simulink model "final2q_all_cases"  (R2024b)
settings: Solver=VariableStepAuto  StartTime=0.0  StopTime=10  RelTol=1e-3
undefined symbols (not defined in the file): Down, Up
libraries: spsSeriesRLCBranchLib x30, spsDCVoltageSourceLib x12, spsIGBTDiodeLib x12, spsVoltageMeasurementLib x12, spsCurrentMeasurementLib x6, slpidlib x2, eePwmGenerator x2, sps_lib x1
settings Model: Creator=jmy  LastModifiedBy=Eng.Abd-Elrhman Saad

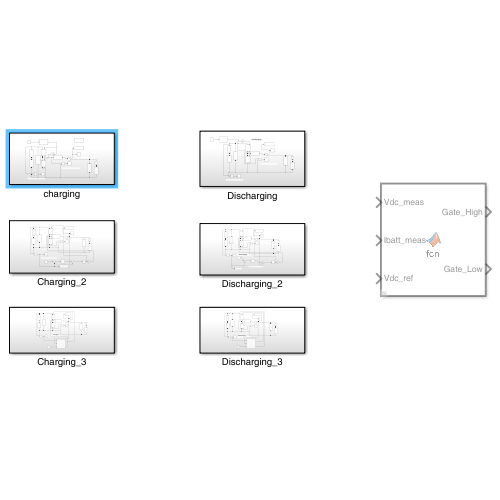
[thumbnail: Simulink's stored preview of the top-level diagram]
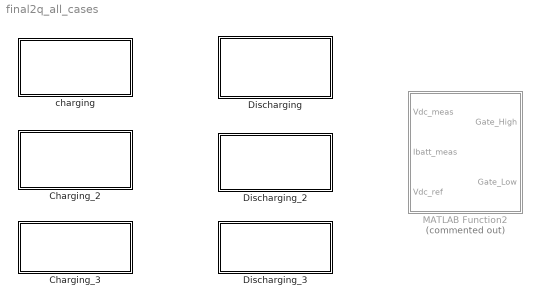
== system final2q_all_cases ==
  Charging_2 : Subsystem
  Charging_3 : Subsystem
  Discharging : Subsystem
  Discharging_2 : Subsystem
  Discharging_3 : Subsystem
  MATLAB Function2 : MATLAB Function  Commented=on  TreatAsAtomicUnit=on
  charging : Subsystem

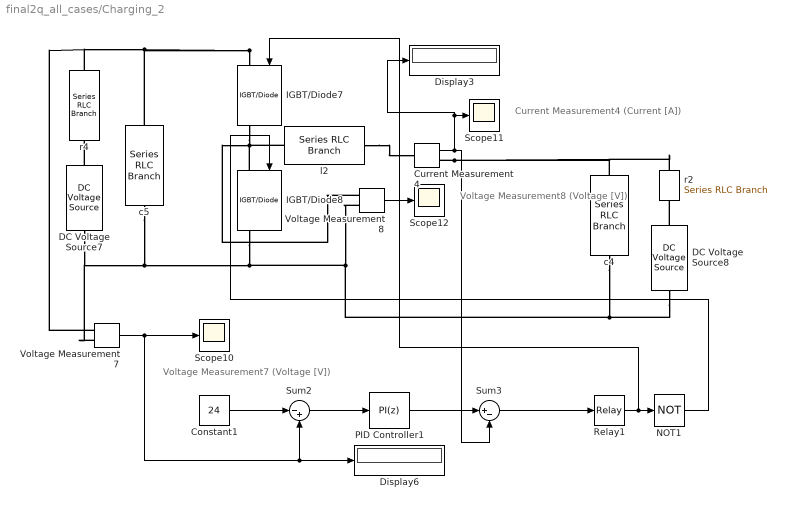
== system final2q_all_cases/Charging_2 ==
  note: Voltage Measurement7 (Voltage [V])
  note: Current Measurement4 (Current [A])
  note: Voltage Measurement8 (Voltage [V])
  Constant1 : Constant  Value=24
  Current Measurement4 : spsCurrentMeasurementLib/Current Measurement  PhasorSimulation=off  OutputType=Complex  PSBequivalent=0
  DC Voltage Source7 : spsDCVoltageSourceLib/DC Voltage Source  Amplitude=26  Measurements=None
  DC Voltage Source8 : spsDCVoltageSourceLib/DC Voltage Source  Amplitude=18.5  Measurements=None
  Display3 : Display
  Display6 : Display
  IGBT/Diode7 : spsIGBTDiodeLib/IGBT//Diode  Ron=1e-3  Rs=1e5  Cs=inf  Measurements=on
  IGBT/Diode8 : spsIGBTDiodeLib/IGBT//Diode  Ron=1e-3  Rs=1e5  Cs=inf  Measurements=on
  NOT1 : Logic  Operator=NOT  IconShape=distinctive  AllPortsSameDT=off  OutDataTypeStr=boolean
  PID Controller1 : slpidlib/PID Controller  Controller=PI  Form=Parallel  TimeDomain=Discrete-time  UseExternalTs=off  SampleTime=-1  IntegratorMethod=Forward Euler  FilterMethod=Forward Euler  ControllerParametersSource=internal  P=0.1  I=10  UseKiTs=off  D=0  UseExternalDerivativeSource=off  N=100  UseFilter=on  TunerSelectOption=Transfer Function Based (PID Tuner App)  InitialConditionSource=internal  InitialConditionForIntegrator=0  InitialConditionForFilter=0  DifferentiatorICPrevScaledInput=0  ExternalReset=none  TrackingMode=off  Kt=1  LimitOutput=on  SatLimitsSource=internal  UpperSaturationLimit=3.1  LowerSaturationLimit=-10  LinearizeAsGain=off  AntiWindupMode=none  Kb=1  LimitIntegrator=off  UpperIntegratorSaturationLimit=inf  LowerIntegratorSaturationLimit=-inf  POutMin=[]  POutMax=[]  IOutMin=[]  IOutMax=[]  DOutMin=[]  DOutMax=[]  NOutMin=[]  NOutMax=[]  SumOutMin=[]  SumOutMax=[]  SaturationOutMin=[]  SaturationOutMax=[]  PParamMin=[]  PParamMax=[]  IParamMin=[]  IParamMax=[]  DParamMin=[]  DParamMax=[]  NParamMin=[]  NParamMax=[]  KbParamMin=[]  KbParamMax=[]  KtParamMin=[]  KtParamMax=[]  KbOutMin=[]  KbOutMax=[]  KtOutMin=[]  KtOutMax=[]  IntegratorOutMin=[]  IntegratorOutMax=[]  FilterOutMin=[]  FilterOutMax=[]  SumI1OutMin=[]  SumI1OutMax=[]  SumI2OutMin=[]  SumI2OutMax=[]  SumI3OutMin=[]  SumI3OutMax=[]  SumI4OutMin=[]  SumI4OutMax=[]  SumDOutMin=[]  SumDOutMax=[]  DifferentiatorOutMin=[]  DifferentiatorOutMax=[]  FilterDiffOutCoefMin=[]  FilterDiffOutCoefMax=[]  ReciprocalOutMin=[]  ReciprocalOutMax=[]  SumDenOutMin=[]  SumDenOutMax=[]  SumNumOutMin=[]  SumNumOutMax=[]  DivideOutMin=[]  DivideOutMax=[]  UdiffTsProdOutMin=[]  UdiffTsProdOutMax=[]  NTsProdOutMin=[]  NTsProdOutMax=[]  UintegralTsProdOutMin=[]  UintegralTsProdOutMax=[]  UngainTsProdOutMin=[]  UngainTsProdOutMax=[]  ClampingZeroOutDataTypeStr=Inherit: Inherit via back propagation  ClampingZeroOutMin=[]  ClampingZeroOutMax=[]  FilterDenConstantOutDataTypeStr=Inherit: Inherit via back propagation  FilterDenConstantOutMin=[]  FilterDenConstantOutMax=[]  PCopyOutDataTypeStr=Inherit: Inherit via back propagation  PCopyOutMin=[]  PCopyOutMax=[]  NCopyOutDataTypeStr=Inherit: Inherit via back propagation  NCopyOutMin=[]  NCopyOutMax=[]  IntegratorContinuousStateAttributes=''  IntegratorStateMustResolveToSignalObject=off  IntegratorRTWStateStorageClass=Auto  FilterContinuousStateAttributes=''  FilterStateMustResolveToSignalObject=off  FilterRTWStateStorageClass=Auto  ParallelPVariant=InternalParameters  IdealPVariant=Disabled  IVariant=InternalParameters  DVariant=Disabled  IntegratorVariant=Discrete  SatVariant=Enabled  AWVariant=Passthrough  PCopyVariant=Disabled  TRVariant=Disabled  FdbkBlocksVariant=Forward  IdealPFdbkVariant=Disabled  SatFdbkVariant=Disabled  DerivativeFilterVariant=Disabled  NVariant=Disabled  NCopyVariant=Disabled_SignalSpec  FilterICVariant=Disabled  IntegratorICVariant=InternalICs  ExternalResetVariant=Disabled  TRSumVariant=Passthrough  SumFdbkVariant=Disabled  SumVariant=Sum_PI  TsampFilterVariant=InternalTs  TsampNgainVariant=Passthrough  TsampIntegralVariant=Disabled_SignalSpec  ExternalSaturationOutDataTypeStr=Inherit: Same as second input  DerivativeSourceVariant=Disabled  PreIntVariant=InternalPreInt
  Relay1 : Relay  OnSwitchValue=0.5  OffSwitchValue=-0.5
  Scope10 : Scope
  Scope11 : Scope
  Scope12 : Scope
  Sum2 : Sum  Inputs=|-+
  Sum3 : Sum  Inputs=|+-
  Voltage Measurement7 : spsVoltageMeasurementLib/Voltage Measurement  PhasorSimulation=off  OutputType=Complex  PSBequivalent=0
  Voltage Measurement8 : spsVoltageMeasurementLib/Voltage Measurement  PhasorSimulation=off  OutputType=Complex  PSBequivalent=0
  c4 : spsSeriesRLCBranchLib/Series RLC Branch  LConnTagsString=__new0  RConnTagsString=__new0  BranchType=C  Resistance=1  Inductance=400e-6  SetiL0=off  InitialCurrent=0  Capacitance=100e-6  Setx0=off  InitialVoltage=0  Measurements=None
  c5 : spsSeriesRLCBranchLib/Series RLC Branch  LConnTagsString=__new0  RConnTagsString=__new0  BranchType=C  Resistance=1  Inductance=400e-6  SetiL0=off  InitialCurrent=0  Capacitance=220e-6  Setx0=off  InitialVoltage=0  Measurements=None
  l2 : spsSeriesRLCBranchLib/Series RLC Branch  LConnTagsString=__new0  RConnTagsString=__new0  BranchType=L  Resistance=1  Inductance=400e-6  SetiL0=off  InitialCurrent=0  Capacitance=1e-6  Setx0=off  InitialVoltage=0  Measurements=None
  r2 : spsSeriesRLCBranchLib/Series RLC Branch  LConnTagsString=__new0  RConnTagsString=__new0  BranchType=R  Resistance=0.0001  Inductance=400e-6  SetiL0=off  InitialCurrent=0  Capacitance=220e-6  Setx0=off  InitialVoltage=0  Measurements=None
  r4 : spsSeriesRLCBranchLib/Series RLC Branch  LConnTagsString=__new0  RConnTagsString=__new0  BranchType=R  Resistance=0.0001  Inductance=400e-6  SetiL0=off  InitialCurrent=0  Capacitance=220e-6  Setx0=off  InitialVoltage=0  Measurements=None
  wires:
  Voltage Measurement7/1 -> Scope10/1, Sum2/2, Display6/1
  Relay1/1 -> NOT1/1, IGBT/Diode7/1
  Voltage Measurement8/1 -> Scope12/1
  Constant1/1 -> Sum2/1
  Current Measurement4/1 -> Sum3/2, Display3/1, Scope11/1
  Sum3/1 -> Relay1/1
  NOT1/1 -> IGBT/Diode8/1
  Sum2/1 -> PID Controller1/1
  PID Controller1/1 -> Sum3/1
  connections:
  IGBT/Diode7/LConn1 -- r4/LConn1 -- Voltage Measurement7/LConn1 -- c5/LConn1
  DC Voltage Source8/LConn1 -- c4/RConn1 -- Voltage Measurement8/LConn2 -- Voltage Measurement7/LConn2 -- DC Voltage Source7/LConn1 -- c5/RConn1 -- IGBT/Diode8/RConn1
  DC Voltage Source8/RConn1 -- r2/RConn1
  l2/LConn1 -- IGBT/Diode8/LConn1 -- IGBT/Diode7/RConn1 -- Voltage Measurement8/LConn1
  Current Measurement4/RConn1 -- r2/LConn1 -- c4/LConn1
  l2/RConn1 -- Current Measurement4/LConn1
  DC Voltage Source7/RConn1 -- r4/RConn1

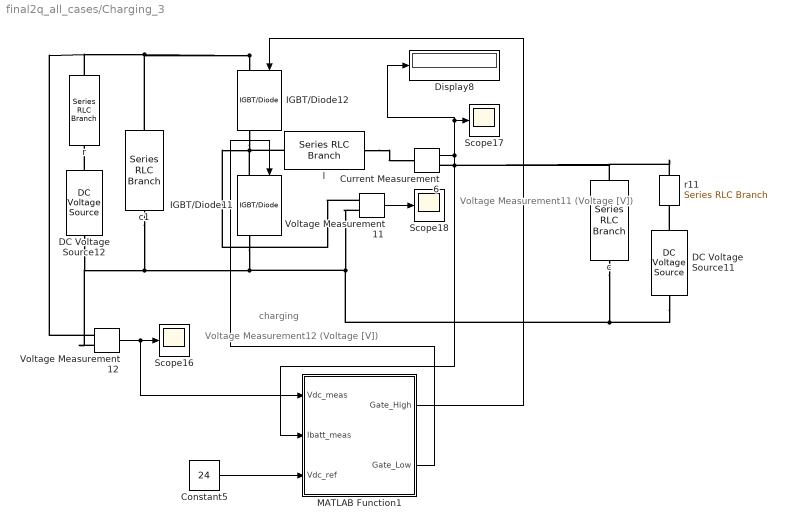
== system final2q_all_cases/Charging_3 ==
  note: charging
  note: Voltage Measurement12 (Voltage [V])
  note: Voltage Measurement11 (Voltage [V])
  Constant5 : Constant  Value=24
  Current Measurement6 : spsCurrentMeasurementLib/Current Measurement  PhasorSimulation=off  OutputType=Complex  PSBequivalent=0
  DC Voltage Source11 : spsDCVoltageSourceLib/DC Voltage Source  Amplitude=18.5  Measurements=None
  DC Voltage Source12 : spsDCVoltageSourceLib/DC Voltage Source  Amplitude=26  Measurements=None
  Display8 : Display
  IGBT/Diode11 : spsIGBTDiodeLib/IGBT//Diode  Ron=1e-3  Rs=1e5  Cs=inf  Measurements=on
  IGBT/Diode12 : spsIGBTDiodeLib/IGBT//Diode  Ron=1e-3  Rs=1e5  Cs=inf  Measurements=on
  MATLAB Function1 : MATLAB Function  TreatAsAtomicUnit=on
  Scope16 : Scope
  Scope17 : Scope
  Scope18 : Scope
  Voltage Measurement11 : spsVoltageMeasurementLib/Voltage Measurement  PhasorSimulation=off  OutputType=Complex  PSBequivalent=0
  Voltage Measurement12 : spsVoltageMeasurementLib/Voltage Measurement  PhasorSimulation=off  OutputType=Complex  PSBequivalent=0
  c : spsSeriesRLCBranchLib/Series RLC Branch  LConnTagsString=__new0  RConnTagsString=__new0  BranchType=C  Resistance=1  Inductance=400e-6  SetiL0=off  InitialCurrent=0  Capacitance=100e-6  Setx0=off  InitialVoltage=0  Measurements=None
  c1 : spsSeriesRLCBranchLib/Series RLC Branch  LConnTagsString=__new0  RConnTagsString=__new0  BranchType=C  Resistance=1  Inductance=400e-6  SetiL0=off  InitialCurrent=0  Capacitance=220e-6  Setx0=off  InitialVoltage=0  Measurements=None
  l : spsSeriesRLCBranchLib/Series RLC Branch  LConnTagsString=__new0  RConnTagsString=__new0  BranchType=L  Resistance=1  Inductance=400e-6  SetiL0=off  InitialCurrent=0  Capacitance=1e-6  Setx0=off  InitialVoltage=0  Measurements=None
  r : spsSeriesRLCBranchLib/Series RLC Branch  LConnTagsString=__new0  RConnTagsString=__new0  BranchType=R  Resistance=0.0001  Inductance=400e-6  SetiL0=off  InitialCurrent=0  Capacitance=220e-6  Setx0=off  InitialVoltage=0  Measurements=None
  r11 : spsSeriesRLCBranchLib/Series RLC Branch  LConnTagsString=__new0  RConnTagsString=__new0  BranchType=R  Resistance=0.0001  Inductance=400e-6  SetiL0=off  InitialCurrent=0  Capacitance=220e-6  Setx0=off  InitialVoltage=0  Measurements=None
  wires:
  Constant5/1 -> MATLAB Function1/3(Vdc_ref)
  Voltage Measurement12/1 -> Scope16/1, MATLAB Function1/1(Vdc_meas)
  MATLAB Function1/2(Gate_Low) -> IGBT/Diode11/1
  MATLAB Function1/1(Gate_High) -> IGBT/Diode12/1
  Current Measurement6/1 -> MATLAB Function1/2(Ibatt_meas), Display8/1, Scope17/1
  Voltage Measurement11/1 -> Scope18/1
  connections:
  IGBT/Diode12/LConn1 -- r/LConn1 -- Voltage Measurement12/LConn1 -- c1/LConn1
  DC Voltage Source11/LConn1 -- Voltage Measurement12/LConn2 -- DC Voltage Source12/LConn1 -- c1/RConn1 -- IGBT/Diode11/RConn1 -- Voltage Measurement11/LConn2 -- c/RConn1
  DC Voltage Source12/RConn1 -- r/RConn1
  Current Measurement6/RConn1 -- r11/LConn1 -- c/LConn1
  l/LConn1 -- IGBT/Diode11/LConn1 -- IGBT/Diode12/RConn1 -- Voltage Measurement11/LConn1
  l/RConn1 -- Current Measurement6/LConn1
  DC Voltage Source11/RConn1 -- r11/RConn1

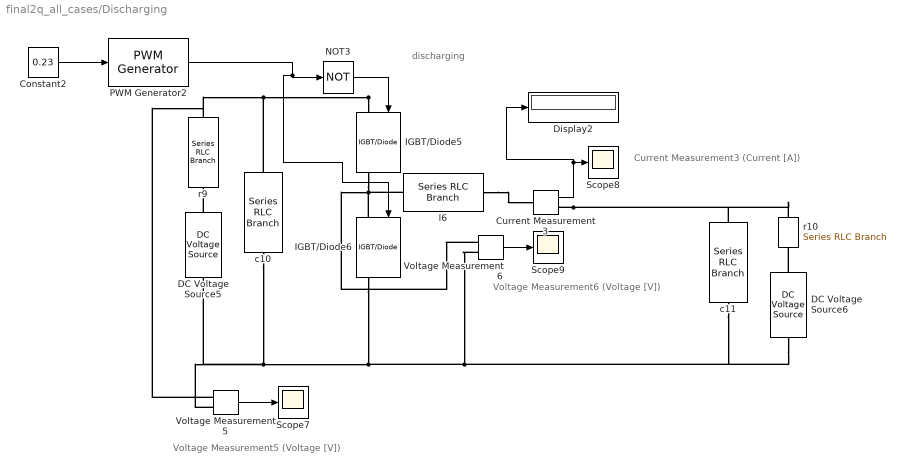
== system final2q_all_cases/Discharging ==
  note: discharging
  note: Voltage Measurement5 (Voltage [V])
  note: Current Measurement3 (Current [A])
  note: Voltage Measurement6 (Voltage [V])
  Constant2 : Constant  Value=0.23
  Current Measurement3 : spsCurrentMeasurementLib/Current Measurement  PhasorSimulation=off  OutputType=Complex  PSBequivalent=0
  DC Voltage Source5 : spsDCVoltageSourceLib/DC Voltage Source  Amplitude=22  Measurements=None
  DC Voltage Source6 : spsDCVoltageSourceLib/DC Voltage Source  Amplitude=18.5  Measurements=None
  Display2 : Display
  IGBT/Diode5 : spsIGBTDiodeLib/IGBT//Diode  Ron=1e-3  Rs=1e5  Cs=inf  Measurements=on
  IGBT/Diode6 : spsIGBTDiodeLib/IGBT//Diode  Ron=1e-3  Rs=1e5  Cs=inf  Measurements=on
  NOT3 : Logic  Operator=NOT  IconShape=distinctive  AllPortsSameDT=off  OutDataTypeStr=boolean
  PWM Generator2 : eePwmGenerator/PWM Generator  CarrCount=Up-Down  Tper=0.001  Tdelay=0  Ts=5e-5
  Scope7 : Scope
  Scope8 : Scope
  Scope9 : Scope
  Voltage Measurement5 : spsVoltageMeasurementLib/Voltage Measurement  PhasorSimulation=off  OutputType=Complex  PSBequivalent=0
  Voltage Measurement6 : spsVoltageMeasurementLib/Voltage Measurement  PhasorSimulation=off  OutputType=Complex  PSBequivalent=0
  c10 : spsSeriesRLCBranchLib/Series RLC Branch  LConnTagsString=__new0  RConnTagsString=__new0  BranchType=C  Resistance=1  Inductance=400e-6  SetiL0=off  InitialCurrent=0  Capacitance=220e-6  Setx0=off  InitialVoltage=0  Measurements=None
  c11 : spsSeriesRLCBranchLib/Series RLC Branch  LConnTagsString=__new0  RConnTagsString=__new0  BranchType=C  Resistance=1  Inductance=400e-6  SetiL0=off  InitialCurrent=0  Capacitance=100e-6  Setx0=off  InitialVoltage=0  Measurements=None
  l6 : spsSeriesRLCBranchLib/Series RLC Branch  LConnTagsString=__new0  RConnTagsString=__new0  BranchType=L  Resistance=1  Inductance=400e-6  SetiL0=off  InitialCurrent=0  Capacitance=1e-6  Setx0=off  InitialVoltage=0  Measurements=None
  r10 : spsSeriesRLCBranchLib/Series RLC Branch  LConnTagsString=__new0  RConnTagsString=__new0  BranchType=R  Resistance=0.0001  Inductance=400e-6  SetiL0=off  InitialCurrent=0  Capacitance=220e-6  Setx0=off  InitialVoltage=0  Measurements=None
  r9 : spsSeriesRLCBranchLib/Series RLC Branch  LConnTagsString=__new0  RConnTagsString=__new0  BranchType=R  Resistance=0.0001  Inductance=400e-6  SetiL0=off  InitialCurrent=0  Capacitance=220e-6  Setx0=off  InitialVoltage=0  Measurements=None
  wires:
  Voltage Measurement6/1 -> Scope9/1
  PWM Generator2/1 -> IGBT/Diode6/1, NOT3/1
  Current Measurement3/1 -> Display2/1, Scope8/1
  NOT3/1 -> IGBT/Diode5/1
  Voltage Measurement5/1 -> Scope7/1
  Constant2/1 -> PWM Generator2/1
  connections:
  IGBT/Diode5/LConn1 -- r9/LConn1 -- Voltage Measurement5/LConn1 -- c10/LConn1
  l6/RConn1 -- Current Measurement3/LConn1
  IGBT/Diode6/RConn1 -- c10/RConn1 -- Voltage Measurement5/LConn2 -- DC Voltage Source5/LConn1 -- Voltage Measurement6/LConn2 -- c11/RConn1 -- DC Voltage Source6/LConn1
  DC Voltage Source5/RConn1 -- r9/RConn1
  IGBT/Diode6/LConn1 -- IGBT/Diode5/RConn1 -- Voltage Measurement6/LConn1 -- l6/LConn1
  DC Voltage Source6/RConn1 -- r10/RConn1
  Current Measurement3/RConn1 -- r10/LConn1 -- c11/LConn1

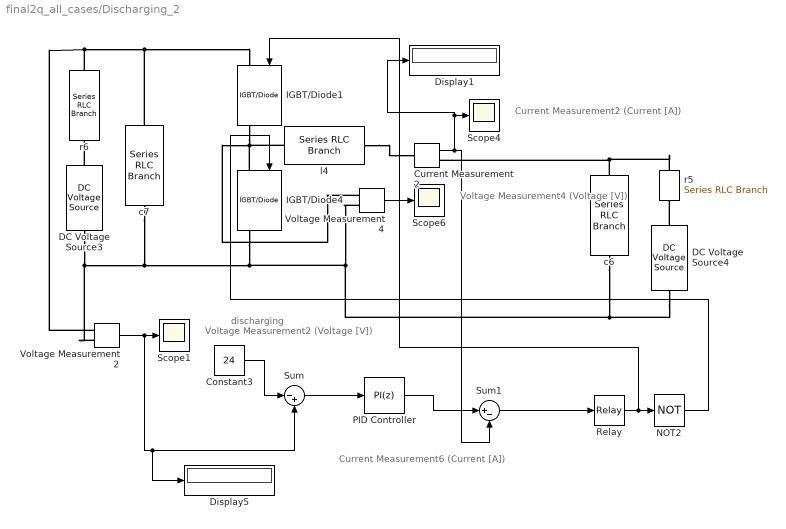
== system final2q_all_cases/Discharging_2 ==
  note: discharging
  note: Voltage Measurement2 (Voltage [V])
  note: Current Measurement6 (Current [A])
  note: Current Measurement2 (Current [A])
  note: Voltage Measurement4 (Voltage [V])
  Constant3 : Constant  Value=24
  Current Measurement2 : spsCurrentMeasurementLib/Current Measurement  PhasorSimulation=off  OutputType=Complex  PSBequivalent=0
  DC Voltage Source3 : spsDCVoltageSourceLib/DC Voltage Source  Amplitude=22  Measurements=None
  DC Voltage Source4 : spsDCVoltageSourceLib/DC Voltage Source  Amplitude=18.5  Measurements=None
  Display1 : Display
  Display5 : Display
  IGBT/Diode1 : spsIGBTDiodeLib/IGBT//Diode  Ron=1e-3  Rs=1e5  Cs=inf  Measurements=on
  IGBT/Diode4 : spsIGBTDiodeLib/IGBT//Diode  Ron=1e-3  Rs=1e5  Cs=inf  Measurements=on
  NOT2 : Logic  Operator=NOT  IconShape=distinctive  AllPortsSameDT=off  OutDataTypeStr=boolean
  PID Controller : slpidlib/PID Controller  Controller=PI  Form=Parallel  TimeDomain=Discrete-time  UseExternalTs=off  SampleTime=-1  IntegratorMethod=Forward Euler  FilterMethod=Forward Euler  ControllerParametersSource=internal  P=0.1  I=10  UseKiTs=off  D=0  UseExternalDerivativeSource=off  N=100  UseFilter=on  TunerSelectOption=Transfer Function Based (PID Tuner App)  InitialConditionSource=internal  InitialConditionForIntegrator=0  InitialConditionForFilter=0  DifferentiatorICPrevScaledInput=0  ExternalReset=none  TrackingMode=off  Kt=1  LimitOutput=on  SatLimitsSource=internal  UpperSaturationLimit=3.1  LowerSaturationLimit=-10  LinearizeAsGain=off  AntiWindupMode=none  Kb=1  LimitIntegrator=off  UpperIntegratorSaturationLimit=inf  LowerIntegratorSaturationLimit=-inf  POutMin=[]  POutMax=[]  IOutMin=[]  IOutMax=[]  DOutMin=[]  DOutMax=[]  NOutMin=[]  NOutMax=[]  SumOutMin=[]  SumOutMax=[]  SaturationOutMin=[]  SaturationOutMax=[]  PParamMin=[]  PParamMax=[]  IParamMin=[]  IParamMax=[]  DParamMin=[]  DParamMax=[]  NParamMin=[]  NParamMax=[]  KbParamMin=[]  KbParamMax=[]  KtParamMin=[]  KtParamMax=[]  KbOutMin=[]  KbOutMax=[]  KtOutMin=[]  KtOutMax=[]  IntegratorOutMin=[]  IntegratorOutMax=[]  FilterOutMin=[]  FilterOutMax=[]  SumI1OutMin=[]  SumI1OutMax=[]  SumI2OutMin=[]  SumI2OutMax=[]  SumI3OutMin=[]  SumI3OutMax=[]  SumI4OutMin=[]  SumI4OutMax=[]  SumDOutMin=[]  SumDOutMax=[]  DifferentiatorOutMin=[]  DifferentiatorOutMax=[]  FilterDiffOutCoefMin=[]  FilterDiffOutCoefMax=[]  ReciprocalOutMin=[]  ReciprocalOutMax=[]  SumDenOutMin=[]  SumDenOutMax=[]  SumNumOutMin=[]  SumNumOutMax=[]  DivideOutMin=[]  DivideOutMax=[]  UdiffTsProdOutMin=[]  UdiffTsProdOutMax=[]  NTsProdOutMin=[]  NTsProdOutMax=[]  UintegralTsProdOutMin=[]  UintegralTsProdOutMax=[]  UngainTsProdOutMin=[]  UngainTsProdOutMax=[]  ClampingZeroOutDataTypeStr=Inherit: Inherit via back propagation  ClampingZeroOutMin=[]  ClampingZeroOutMax=[]  FilterDenConstantOutDataTypeStr=Inherit: Inherit via back propagation  FilterDenConstantOutMin=[]  FilterDenConstantOutMax=[]  PCopyOutDataTypeStr=Inherit: Inherit via back propagation  PCopyOutMin=[]  PCopyOutMax=[]  NCopyOutDataTypeStr=Inherit: Inherit via back propagation  NCopyOutMin=[]  NCopyOutMax=[]  IntegratorContinuousStateAttributes=''  IntegratorStateMustResolveToSignalObject=off  IntegratorRTWStateStorageClass=Auto  FilterContinuousStateAttributes=''  FilterStateMustResolveToSignalObject=off  FilterRTWStateStorageClass=Auto  ParallelPVariant=InternalParameters  IdealPVariant=Disabled  IVariant=InternalParameters  DVariant=Disabled  IntegratorVariant=Discrete  SatVariant=Enabled  AWVariant=Passthrough  PCopyVariant=Disabled  TRVariant=Disabled  FdbkBlocksVariant=Forward  IdealPFdbkVariant=Disabled  SatFdbkVariant=Disabled  DerivativeFilterVariant=Disabled  NVariant=Disabled  NCopyVariant=Disabled_SignalSpec  FilterICVariant=Disabled  IntegratorICVariant=InternalICs  ExternalResetVariant=Disabled  TRSumVariant=Passthrough  SumFdbkVariant=Disabled  SumVariant=Sum_PI  TsampFilterVariant=InternalTs  TsampNgainVariant=Passthrough  TsampIntegralVariant=Disabled_SignalSpec  ExternalSaturationOutDataTypeStr=Inherit: Same as second input  DerivativeSourceVariant=Disabled  PreIntVariant=InternalPreInt
  Relay : Relay  OnSwitchValue=0.5  OffSwitchValue=-0.5
  Scope1 : Scope
  Scope4 : Scope
  Scope6 : Scope
  Sum : Sum  Inputs=|-+
  Sum1 : Sum  Inputs=|+-
  Voltage Measurement2 : spsVoltageMeasurementLib/Voltage Measurement  PhasorSimulation=off  OutputType=Complex  PSBequivalent=0
  Voltage Measurement4 : spsVoltageMeasurementLib/Voltage Measurement  PhasorSimulation=off  OutputType=Complex  PSBequivalent=0
  c6 : spsSeriesRLCBranchLib/Series RLC Branch  LConnTagsString=__new0  RConnTagsString=__new0  BranchType=C  Resistance=1  Inductance=400e-6  SetiL0=off  InitialCurrent=0  Capacitance=100e-6  Setx0=off  InitialVoltage=0  Measurements=None
  c7 : spsSeriesRLCBranchLib/Series RLC Branch  LConnTagsString=__new0  RConnTagsString=__new0  BranchType=C  Resistance=1  Inductance=400e-6  SetiL0=off  InitialCurrent=0  Capacitance=220e-6  Setx0=off  InitialVoltage=0  Measurements=None
  l4 : spsSeriesRLCBranchLib/Series RLC Branch  LConnTagsString=__new0  RConnTagsString=__new0  BranchType=L  Resistance=1  Inductance=400e-6  SetiL0=off  InitialCurrent=0  Capacitance=1e-6  Setx0=off  InitialVoltage=0  Measurements=None
  r5 : spsSeriesRLCBranchLib/Series RLC Branch  LConnTagsString=__new0  RConnTagsString=__new0  BranchType=R  Resistance=0.0001  Inductance=400e-6  SetiL0=off  InitialCurrent=0  Capacitance=220e-6  Setx0=off  InitialVoltage=0  Measurements=None
  r6 : spsSeriesRLCBranchLib/Series RLC Branch  LConnTagsString=__new0  RConnTagsString=__new0  BranchType=R  Resistance=0.0001  Inductance=400e-6  SetiL0=off  InitialCurrent=0  Capacitance=220e-6  Setx0=off  InitialVoltage=0  Measurements=None
  wires:
  Voltage Measurement2/1 -> Display5/1, Sum/2, Scope1/1
  Current Measurement2/1 -> Scope4/1, Display1/1, Sum1/2
  NOT2/1 -> IGBT/Diode4/1
  Relay/1 -> IGBT/Diode1/1, NOT2/1
  Sum1/1 -> Relay/1
  Constant3/1 -> Sum/1
  Sum/1 -> PID Controller/1
  PID Controller/1 -> Sum1/1
  Voltage Measurement4/1 -> Scope6/1
  connections:
  DC Voltage Source3/RConn1 -- r6/RConn1
  Voltage Measurement2/LConn2 -- IGBT/Diode4/RConn1 -- Voltage Measurement4/LConn2 -- DC Voltage Source4/LConn1 -- c6/RConn1 -- c7/RConn1 -- DC Voltage Source3/LConn1
  DC Voltage Source4/RConn1 -- r5/RConn1
  r5/LConn1 -- Current Measurement2/RConn1 -- c6/LConn1
  IGBT/Diode4/LConn1 -- l4/LConn1 -- Voltage Measurement4/LConn1 -- IGBT/Diode1/RConn1
  r6/LConn1 -- Voltage Measurement2/LConn1 -- IGBT/Diode1/LConn1 -- c7/LConn1
  l4/RConn1 -- Current Measurement2/LConn1

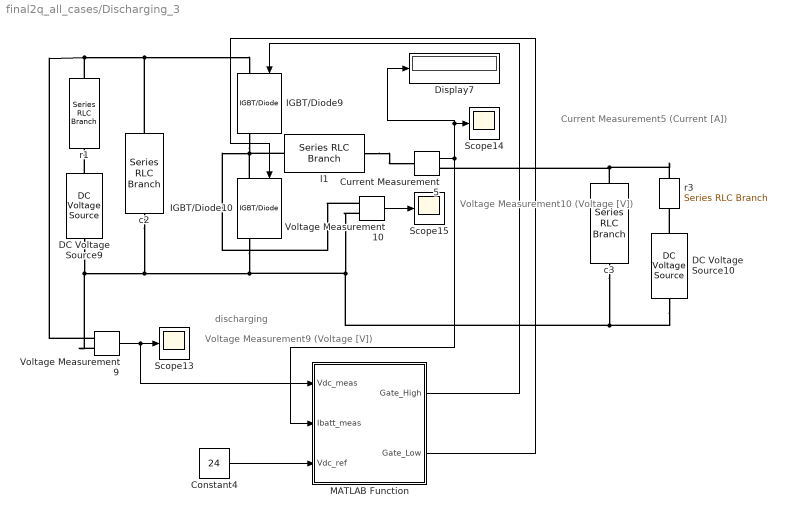
== system final2q_all_cases/Discharging_3 ==
  note: discharging
  note: Voltage Measurement9 (Voltage [V])
  note: Current Measurement5 (Current [A])
  note: Voltage Measurement10 (Voltage [V])
  Constant4 : Constant  Value=24
  Current Measurement5 : spsCurrentMeasurementLib/Current Measurement  PhasorSimulation=off  OutputType=Complex  PSBequivalent=0
  DC Voltage Source10 : spsDCVoltageSourceLib/DC Voltage Source  Amplitude=18.5  Measurements=None
  DC Voltage Source9 : spsDCVoltageSourceLib/DC Voltage Source  Amplitude=23.5  Measurements=None
  Display7 : Display
  IGBT/Diode10 : spsIGBTDiodeLib/IGBT//Diode  Ron=1e-3  Rs=1e5  Cs=inf  Measurements=on
  IGBT/Diode9 : spsIGBTDiodeLib/IGBT//Diode  Ron=1e-3  Rs=1e5  Cs=inf  Measurements=on
  MATLAB Function : MATLAB Function  TreatAsAtomicUnit=on
  Scope13 : Scope
  Scope14 : Scope
  Scope15 : Scope
  Voltage Measurement10 : spsVoltageMeasurementLib/Voltage Measurement  PhasorSimulation=off  OutputType=Complex  PSBequivalent=0
  Voltage Measurement9 : spsVoltageMeasurementLib/Voltage Measurement  PhasorSimulation=off  OutputType=Complex  PSBequivalent=0
  c2 : spsSeriesRLCBranchLib/Series RLC Branch  LConnTagsString=__new0  RConnTagsString=__new0  BranchType=C  Resistance=1  Inductance=400e-6  SetiL0=off  InitialCurrent=0  Capacitance=220e-6  Setx0=off  InitialVoltage=0  Measurements=None
  c3 : spsSeriesRLCBranchLib/Series RLC Branch  LConnTagsString=__new0  RConnTagsString=__new0  BranchType=C  Resistance=1  Inductance=400e-6  SetiL0=off  InitialCurrent=0  Capacitance=100e-6  Setx0=off  InitialVoltage=0  Measurements=None
  l1 : spsSeriesRLCBranchLib/Series RLC Branch  LConnTagsString=__new0  RConnTagsString=__new0  BranchType=L  Resistance=1  Inductance=400e-6  SetiL0=off  InitialCurrent=0  Capacitance=1e-6  Setx0=off  InitialVoltage=0  Measurements=None
  r1 : spsSeriesRLCBranchLib/Series RLC Branch  LConnTagsString=__new0  RConnTagsString=__new0  BranchType=R  Resistance=0.0001  Inductance=400e-6  SetiL0=off  InitialCurrent=0  Capacitance=220e-6  Setx0=off  InitialVoltage=0  Measurements=None
  r3 : spsSeriesRLCBranchLib/Series RLC Branch  LConnTagsString=__new0  RConnTagsString=__new0  BranchType=R  Resistance=0.0001  Inductance=400e-6  SetiL0=off  InitialCurrent=0  Capacitance=220e-6  Setx0=off  InitialVoltage=0  Measurements=None
  wires:
  MATLAB Function/1(Gate_High) -> IGBT/Diode9/1
  Constant4/1 -> MATLAB Function/3(Vdc_ref)
  Current Measurement5/1 -> Scope14/1, Display7/1, MATLAB Function/2(Ibatt_meas)
  Voltage Measurement9/1 -> MATLAB Function/1(Vdc_meas), Scope13/1
  MATLAB Function/2(Gate_Low) -> IGBT/Diode10/1
  Voltage Measurement10/1 -> Scope15/1
  connections:
  IGBT/Diode10/LConn1 -- l1/LConn1 -- Voltage Measurement10/LConn1 -- IGBT/Diode9/RConn1
  r3/LConn1 -- Current Measurement5/RConn1 -- c3/LConn1
  Voltage Measurement9/LConn2 -- DC Voltage Source10/LConn1 -- c3/RConn1 -- Voltage Measurement10/LConn2 -- IGBT/Diode10/RConn1 -- c2/RConn1 -- DC Voltage Source9/LConn1
  DC Voltage Source9/RConn1 -- r1/RConn1
  r1/LConn1 -- IGBT/Diode9/LConn1 -- c2/LConn1 -- Voltage Measurement9/LConn1
  l1/RConn1 -- Current Measurement5/LConn1
  DC Voltage Source10/RConn1 -- r3/RConn1

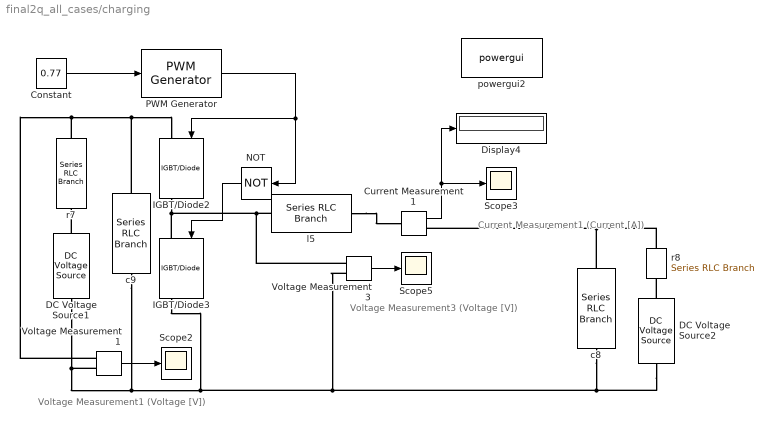
== system final2q_all_cases/charging ==
  note: Voltage Measurement1 (Voltage [V])
  note: Current Measurement1 (Current [A])
  note: Voltage Measurement3 (Voltage [V])
  Constant : Constant  Value=0.77
  Current Measurement1 : spsCurrentMeasurementLib/Current Measurement  PhasorSimulation=off  OutputType=Complex  PSBequivalent=0
  DC Voltage Source1 : spsDCVoltageSourceLib/DC Voltage Source  Amplitude=24  Measurements=None
  DC Voltage Source2 : spsDCVoltageSourceLib/DC Voltage Source  Amplitude=18.5  Measurements=None
  Display4 : Display
  IGBT/Diode2 : spsIGBTDiodeLib/IGBT//Diode  Ron=1e-3  Rs=1e5  Cs=inf  Measurements=on
  IGBT/Diode3 : spsIGBTDiodeLib/IGBT//Diode  Ron=1e-3  Rs=1e5  Cs=inf  Measurements=on
  NOT : Logic  Operator=NOT  IconShape=distinctive  AllPortsSameDT=off  OutDataTypeStr=boolean
  PWM Generator : eePwmGenerator/PWM Generator  CarrCount=Up-Down  Tper=0.001  Tdelay=0  Ts=5e-5
  Scope2 : Scope
  Scope3 : Scope
  Scope5 : Scope
  Voltage Measurement1 : spsVoltageMeasurementLib/Voltage Measurement  PhasorSimulation=off  OutputType=Complex  PSBequivalent=0
  Voltage Measurement3 : spsVoltageMeasurementLib/Voltage Measurement  PhasorSimulation=off  OutputType=Complex  PSBequivalent=0
  c8 : spsSeriesRLCBranchLib/Series RLC Branch  LConnTagsString=__new0  RConnTagsString=__new0  BranchType=C  Resistance=1  Inductance=400e-6  SetiL0=off  InitialCurrent=0  Capacitance=100e-6  Setx0=off  InitialVoltage=0  Measurements=None
  c9 : spsSeriesRLCBranchLib/Series RLC Branch  LConnTagsString=__new0  RConnTagsString=__new0  BranchType=C  Resistance=1  Inductance=400e-6  SetiL0=off  InitialCurrent=0  Capacitance=220e-6  Setx0=off  InitialVoltage=0  Measurements=None
  l5 : spsSeriesRLCBranchLib/Series RLC Branch  LConnTagsString=__new0  RConnTagsString=__new0  BranchType=L  Resistance=1  Inductance=400e-6  SetiL0=off  InitialCurrent=0  Capacitance=1e-6  Setx0=off  InitialVoltage=0  Measurements=None
  powergui2 : sps_lib/powergui  Priority=1  SimulationMode=Discrete  SampleTime=50e-6  frequency=60  Iterations=50  frequencyindice=0  Pbase=100e6  ErrMax=1e-4  UnitsV=kV  UnitsW=MW  buscounter=0  FunctionMessages=off  echomessages=off  EnableUseOfTLC=off  CurrentSourceSwitches=off  DisableSnubberDevices=off  DisableRonSwitches=off  DisableVfSwitches=off  DisplayEquations=off  AutomaticDiscreteSolvers=off  SolverType=Tustin/Backward Euler (TBE)  Interpol=off  ExternalGateDelay=off  methode=off  Ts=100  x0status=blocks  SPID=on  SwTol=0  HookPort=off  NonlinearTolerance=1e-4  nMaxIteration=100  ContinueOnMaxIteration=off  RestoreLinks=warning  ResistiveCurrentMeasurement=off  Frange=[0:2:500]  Ylog=off  Xlog=on  ShowGrid=off  save=off  variable=ZData  structure=0  ZoomFFT=off  StartTime=0.0  cycles=1  DisplayStyle=1  fundamental=60  FreqAxis=off  MaxFrequency=1000  frequencyindicesteady=1  RmsSteady=1  display=off
  r7 : spsSeriesRLCBranchLib/Series RLC Branch  LConnTagsString=__new0  RConnTagsString=__new0  BranchType=R  Resistance=0.0001  Inductance=400e-6  SetiL0=off  InitialCurrent=0  Capacitance=220e-6  Setx0=off  InitialVoltage=0  Measurements=None
  r8 : spsSeriesRLCBranchLib/Series RLC Branch  LConnTagsString=__new0  RConnTagsString=__new0  BranchType=R  Resistance=0.0001  Inductance=400e-6  SetiL0=off  InitialCurrent=0  Capacitance=220e-6  Setx0=off  InitialVoltage=0  Measurements=None
  wires:
  PWM Generator/1 -> IGBT/Diode2/1, NOT/1
  Current Measurement1/1 -> Display4/1, Scope3/1
  Constant/1 -> PWM Generator/1
  Voltage Measurement3/1 -> Scope5/1
  Voltage Measurement1/1 -> Scope2/1
  NOT/1 -> IGBT/Diode3/1
  connections:
  DC Voltage Source2/RConn1 -- r8/RConn1
  IGBT/Diode3/LConn1 -- Voltage Measurement3/LConn1 -- l5/LConn1 -- IGBT/Diode2/RConn1
  r7/LConn1 -- Voltage Measurement1/LConn1 -- c9/LConn1 -- IGBT/Diode2/LConn1
  r8/LConn1 -- c8/LConn1 -- Current Measurement1/RConn1
  Voltage Measurement1/LConn2 -- DC Voltage Source1/LConn1 -- c9/RConn1 -- IGBT/Diode3/RConn1 -- Voltage Measurement3/LConn2 -- c8/RConn1 -- DC Voltage Source2/LConn1
  l5/RConn1 -- Current Measurement1/LConn1
  DC Voltage Source1/RConn1 -- r7/RConn1

== matlab function final2q_all_cases/Charging_3/MATLAB Function1 ==
  data: Vdc_meas input; Gate_High output; Ibatt_meas input; Vdc_ref input; Gate_Low output
function [Gate_High, Gate_Low] = fcn(Vdc_meas, Ibatt_meas, Vdc_ref)
    % --- PART 1: Memory (Persistent Variables) ---
    persistent int_err_v S_high
    if isempty(int_err_v)
        int_err_v = 0;
        S_high = 0;
    end

    % --- Internal Constants ---
    Ts = 5e-5;      % Sampling time (from your powergui)
    h = 0.01;        % Hysteresis band
    Kp_v = 0.1;     % PI Proportional Gain
    Ki_v = 10;      % PI Integral Gain

    % --- PART 2: Outer Loop (Voltage PI Control) ---
    err_v = Vdc_meas - Vdc_ref ;
    int_err_v = int_err_v + err_v * Ts;
    
    % Anti-windup (Clamping the integrator)
    int_err_v = max(min(int_err_v, 5), -5); 
    
    % Calculate the Current Reference (I_ref)
    I_ref = (Kp_v * err_v) + (Ki_v * int_err_v);

    % --- PART 3: Current Saturation (Protection) ---
    % Logic: Charging = Positive (+3.1A max), Discharging = Negative (-10A max)
    I_max_charge = 3.1;   
    I_max_disch  = -10.0; 
    
    % This line is Part 3: It clamps the reference to your hardware limits
    I_ref_sat = max(I_max_disch, min(I_max_charge, I_ref));

    % --- PART 4: Inner Loop (Hysteresis Current Control) ---
    % S_high = 1: Top IGBT ON (Increases current)
    % S_high = 0: Bottom IGBT ON (Decreases current)
    if Ibatt_meas < (I_ref_sat - h)
        S_high = 1;
    elseif Ibatt_meas > (I_ref_sat + h)
        S_high = 0;
    end

    % --- PART 5: Gate Outputs ---
    Gate_High = S_high;
    Gate_Low  = 1 - S_high; % Complementary switching
end

== matlab function final2q_all_cases/Discharging_3/MATLAB Function ==
  data: Vdc_meas input; Gate_High output; Ibatt_meas input; Vdc_ref input; Gate_Low output
function [Gate_High, Gate_Low] = fcn(Vdc_meas, Ibatt_meas, Vdc_ref)
    % --- PART 1: Memory (Persistent Variables) ---
    persistent int_err_v S_high
    if isempty(int_err_v)
        int_err_v = 0;
        S_high = 0;
    end

    % --- Internal Constants ---
    Ts = 5e-5;      % Sampling time (from your powergui)
    h = 0.05;        % Hysteresis band
    Kp_v = 0.1;     % PI Proportional Gain
    Ki_v = 10;      % PI Integral Gain

    % --- PART 2: Outer Loop (Voltage PI Control) ---
    err_v = Vdc_meas - Vdc_ref ;
    int_err_v = int_err_v + err_v * Ts;
    
    % Anti-windup (Clamping the integrator)
    int_err_v = max(min(int_err_v, 5), -5); 
    
    % Calculate the Current Reference (I_ref)
    I_ref = (Kp_v * err_v) + (Ki_v * int_err_v);

    % --- PART 3: Current Saturation (Protection) ---
    % Logic: Charging = Positive (+3.1A max), Discharging = Negative (-10A max)
    I_max_charge = 3.1;   
    I_max_disch  = -10.0; 
    
    % This line is Part 3: It clamps the reference to your hardware limits
    I_ref_sat = max(I_max_disch, min(I_max_charge, I_ref));

    % --- PART 4: Inner Loop (Hysteresis Current Control) ---
    % S_high = 1: Top IGBT ON (Increases current)
    % S_high = 0: Bottom IGBT ON (Decreases current)
    if Ibatt_meas < (I_ref_sat - h)
        S_high = 1;
    elseif Ibatt_meas > (I_ref_sat + h)
        S_high = 0;
    end

    % --- PART 5: Gate Outputs ---
    Gate_High = S_high;
    Gate_Low  = 1 - S_high; % Complementary switching
end

== matlab function final2q_all_cases/MATLAB Function2 ==
  data: Vdc_meas input; Gate_High output; Ibatt_meas input; Vdc_ref input; Gate_Low output
function [Gate_High, Gate_Low] = fcn(Vdc_meas, Ibatt_meas, Vdc_ref)
    % Persistent variables for the PI integrator and switch state
    persistent int_err_v S_high
    if isempty(int_err_v)
        int_err_v = 0;
        S_high = 0;
    end

    % --- Internal Constants ---
    Ts = 5e-5;            % Matches your PowerGUI (50 microseconds)
    h = 0.1;              % Hysteresis band (Fixed at 0.1 Amperes)
    
    % PI Gains
    Kp_v = 1.2;           
    Ki_v = 35;            
    
    % Battery Safety Limits
    % Max charge: 3.1A (Negative) | Max discharge: 10A (Positive)
    I_max_disch = 10.0;
    I_max_charge = -3.1;

    % --- 1. Outer Loop: Voltage PI Control ---
    err_v = Vdc_ref - Vdc_meas;
    
    % Update integrator with anti-windup clamping
    int_err_v = int_err_v + err_v * Ts;
    int_err_v = max(min(int_err_v, 5), -5); 
    
    % Calculate desired current (I_ref)
    I_ref = (Kp_v * err_v) + (Ki_v * int_err_v);

    % Force I_ref to stay within battery specs
    if I_ref > I_max_disch
        I_ref = I_max_disch;
    elseif I_ref < I_max_charge
        I_ref = I_max_charge;
    end

    % --- 2. Inner Loop: Hysteresis Logic ---
    % S_high = 1 -> Top IGBT closed (Increases inductor current)
    % S_high = 0 -> Bottom IGBT closed (Decreases inductor current)
    if Ibatt_meas < (I_ref - h)
        S_high = 1;
    elseif Ibatt_meas > (I_ref + h)
        S_high = 0;
    end

    % --- 3. Final Gate Outputs ---
    Gate_High = S_high;
    Gate_Low  = 1 - S_high; % Complementary signal
endfunction [Gate_High, Gate_Low] = fcn(Vdc_meas, Ibatt_meas, Vdc_ref)
